simulink model "afe_dq_ttype"  (R2026b)
settings: Solver=ode23tb  StopTime=param.sim.simlength  FixedStep=param.sim.tc  MaxStep=param.glb_time.tc
values from neighbouring files (symbols this model uses):
  param = struct()    [init_model.m]
undefined symbols (not defined in the file or in its folder): magnitude
libraries: fl_lib x281, nesl_utility x136, igbt_simple_2th_lib x12, single_phase_transformer_lib x3, discrete_time_low_pass_filter x1, threephase_inductor_lib x1, dclink_for_three_levels x1, three_phase_three_level_ttype_inverter_ideal_switch_based_model x1, three_phase_three_levels_PWM_modulator x1, three_phase_bridge_three_level_ttype_igbt_simple_2th x1, three_phase_voltage_with_frt_emulator_mfcn x1
(part 2 of 8)

== system afe_dq_ttype/afe_dq_mod1/LCL_filter/threephase_vi_measures_stack1 ==
  Bus Creator : BusCreator  Inputs=6
  Current Sensor : fl_lib/Electrical/Electrical Sensors/Current Sensor
  Current Sensor1 : fl_lib/Electrical/Electrical Sensors/Current Sensor
  Current Sensor2 : fl_lib/Electrical/Electrical Sensors/Current Sensor
  Electrical Reference1 : fl_lib/Electrical/Electrical Elements/Electrical Reference
  Gain1 : Gain  Gain=1/param.afe.hw.ubez
  Gain2 : Gain  Gain=1/param.afe.hw.ubez
  Gain3 : Gain  Gain=1/param.afe.hw.ubez
  Gain4 : Gain  Gain=1/param.afe.hw.ibez
  Gain5 : Gain  Gain=1/param.afe.hw.ibez
  Gain6 : Gain  Gain=1/param.afe.hw.ibez
  Selector : Selector  InputPortWidth=6  IndexOptions=Index vector (dialog)  Indices=[1 2 3]  OutputSizes=1  RuntimeRangeChecks=off
  Selector1 : Selector  InputPortWidth=6  IndexOptions=Index vector (dialog)  Indices=[4 5 6]  OutputSizes=1  RuntimeRangeChecks=off
  Voltage Sensor : fl_lib/Electrical/Electrical Sensors/Voltage Sensor
  Voltage Sensor1 : fl_lib/Electrical/Electrical Sensors/Voltage Sensor
  Voltage Sensor2 : fl_lib/Electrical/Electrical Sensors/Voltage Sensor
  ia_grid : nesl_utility/PS-Simulink Converter  PhysicalDomain=network_engine_domain  SubClassName=ps_output  LeftPortType=input  RightPortType=output  PseudoPeriodic=off  Frequencies=[]  VectorFormat=1-D array  Unit=A  AffineConversion=off
  ib_grid : nesl_utility/PS-Simulink Converter  PhysicalDomain=network_engine_domain  SubClassName=ps_output  LeftPortType=input  RightPortType=output  PseudoPeriodic=off  Frequencies=[]  VectorFormat=1-D array  Unit=A  AffineConversion=off
  ic_grid : nesl_utility/PS-Simulink Converter  PhysicalDomain=network_engine_domain  SubClassName=ps_output  LeftPortType=input  RightPortType=output  PseudoPeriodic=off  Frequencies=[]  VectorFormat=1-D array  Unit=A  AffineConversion=off
  ua_grid : nesl_utility/PS-Simulink Converter  PhysicalDomain=network_engine_domain  SubClassName=ps_output  LeftPortType=input  RightPortType=output  PseudoPeriodic=off  Frequencies=[]  VectorFormat=1-D array  Unit=V  AffineConversion=off
  ub_grid : nesl_utility/PS-Simulink Converter  PhysicalDomain=network_engine_domain  SubClassName=ps_output  LeftPortType=input  RightPortType=output  PseudoPeriodic=off  Frequencies=[]  VectorFormat=1-D array  Unit=V  AffineConversion=off
  uc_grid : nesl_utility/PS-Simulink Converter  PhysicalDomain=network_engine_domain  SubClassName=ps_output  LeftPortType=input  RightPortType=output  PseudoPeriodic=off  Frequencies=[]  VectorFormat=1-D array  Unit=V  AffineConversion=off
  Ua : PMIOPort  Side=Left
  ua : PMIOPort  Port=2  Side=Right
  Ub : PMIOPort  Port=3  Side=Left
  ub : PMIOPort  Port=4  Side=Right
  Uc : PMIOPort  Port=5  Side=Left
  uc : PMIOPort  Port=6  Side=Right
  tag scope: ig_abc_pu_mod1=global, ug_abc_pu_mod1=global
  wires:
  Selector1/1 -> [ig_abc_pu_mod1]
  uc_grid/1 -> Gain3/1
  ub_grid/1 -> Gain2/1
  ua_grid/1 -> Gain1/1
  ic_grid/1 -> Gain5/1
  ia_grid/1 -> Gain6/1
  ib_grid/1 -> Gain4/1
  Selector/1 -> [ug_abc_pu_mod1]
  Bus Creator/1 -> Selector1/1, Selector/1  "vi_data"
  Gain1/1 -> Bus Creator/1  "ua_grid_pu"
  Gain2/1 -> Bus Creator/2  "ub_grid_pu"
  Gain3/1 -> Bus Creator/3  "uc_grid_pu"
  Gain6/1 -> Bus Creator/4  "ia_grid_pu"
  Gain4/1 -> Bus Creator/5  "ib_grid_pu"
  Gain5/1 -> Bus Creator/6  "ic_grid_pu"
  connections:
  Current Sensor2/RConn2 -- uc/RConn1
  ic_grid/LConn1 -- Current Sensor2/RConn1
  ia_grid/LConn1 -- Current Sensor/RConn1
  ib_grid/LConn1 -- Current Sensor1/RConn1
  Voltage Sensor2/RConn1 -- uc_grid/LConn1
  Current Sensor1/RConn2 -- ub/RConn1
  Voltage Sensor/LConn1 -- Current Sensor/LConn1 -- Ua/RConn1
  Current Sensor2/LConn1 -- Voltage Sensor2/LConn1 -- Uc/RConn1
  Voltage Sensor1/RConn1 -- ub_grid/LConn1
  Current Sensor/RConn2 -- ua/RConn1
  Voltage Sensor/RConn1 -- ua_grid/LConn1
  Voltage Sensor1/RConn2 -- Voltage Sensor2/RConn2 -- Voltage Sensor/RConn2 -- Electrical Reference1/LConn1
  Voltage Sensor1/LConn1 -- Current Sensor1/LConn1 -- Ub/RConn1

== system afe_dq_ttype/afe_dq_mod1/afe/deadtime_generator_for_ttype ==
  gate_cmds_in : Inport
  Bus Creator : BusCreator  Inputs=3
  dead_time_generator_cmos_simulink_phu : Subsystem  mask{ts=param.glb_time.tc, positive_voltage_rail=15, dead_time=param.glb_time.dead_time_AFE}
      mask prompts: ts "PT1 tau [s]"; positive_voltage_rail "Positive Voltage Rail [V]"; dead_time "DeadTime [s]"
  dead_time_generator_cmos_simulink_phv : Subsystem  mask{ts=param.glb_time.tc, positive_voltage_rail=15, dead_time=param.glb_time.dead_time_AFE}
      mask prompts: ts "PT1 tau [s]"; positive_voltage_rail "Positive Voltage Rail [V]"; dead_time "DeadTime [s]"
  dead_time_generator_cmos_simulink_phw : Subsystem  mask{ts=param.glb_time.tc, positive_voltage_rail=15, dead_time=param.glb_time.dead_time_AFE}
      mask prompts: ts "PT1 tau [s]"; positive_voltage_rail "Positive Voltage Rail [V]"; dead_time "DeadTime [s]"
  gate_cmds_out : Outport
  wires:
  Bus Creator/1 -> gate_cmds_out/1  "gate_cmds"
  dead_time_generator_cmos_simulink_phu/1(cmd_gates) -> Bus Creator/1  "gate_cmds_phu"
  gate_cmds_in/1 -> dead_time_generator_cmos_simulink_phu/1(gate_commands), dead_time_generator_cmos_simulink_phw/1(gate_commands), dead_time_generator_cmos_simulink_phv/1(gate_commands)
  dead_time_generator_cmos_simulink_phw/1(cmd_gates) -> Bus Creator/3  "gate_cmds_phw"
  dead_time_generator_cmos_simulink_phv/1(cmd_gates) -> Bus Creator/2  "gate_cmds_phv"

== system afe_dq_ttype/afe_dq_mod1/afe/ideal_switch_based_three_level_inverter_ttype ==
  gate_commands : Inport
  ideal_switch_based_three_level_inverter_ttype : three_phase_three_level_ttype_inverter_ideal_switch_based_model/ideal_switch_based_three_level_inverter_ttype  Vth=5.5  Ron=1.5e-3  Vdon_diode=2  Rdon_diode=0.15e-3  Csnubber=10e-9  Rsnubber=2200
  uu : PMIOPort  Side=Left
  uv : PMIOPort  Port=2  Side=Left
  udc(+) : PMIOPort  Port=3  Side=Right
  np : PMIOPort  Port=4  Side=Right
  udc(-) : PMIOPort  Port=5  Side=Right
  uw : PMIOPort  Port=6  Side=Left
  wires:
  gate_commands/1 -> ideal_switch_based_three_level_inverter_ttype/1
  connections:
  ideal_switch_based_three_level_inverter_ttype/RConn3 -- udc(-)/RConn1
  uv/RConn1 -- ideal_switch_based_three_level_inverter_ttype/LConn2
  ideal_switch_based_three_level_inverter_ttype/LConn1 -- uu/RConn1
  udc(+)/RConn1 -- ideal_switch_based_three_level_inverter_ttype/RConn1
  ideal_switch_based_three_level_inverter_ttype/LConn3 -- uw/RConn1
  ideal_switch_based_three_level_inverter_ttype/RConn2 -- np/RConn1

== system afe_dq_ttype/afe_dq_mod1/afe/igbt_based_three_level_three_phase_inverter_ttype ==
  gate_commands : Inport
  Bus Selector1 : BusSelector  OutputSignals=igbt_ploss_Q1,igbt_ploss_Q4,igbt_ploss_Q2,igbt_ploss_Q3  OutputAsBus=on
  Bus Selector2 : BusSelector  OutputSignals=diode_ploss_Q4,diode_ploss_Q3,diode_ploss_Q2,diode_ploss_Q1  OutputAsBus=on
  diode_plosses : Scope
      settings: ActiveDisplayYMinimum=-84.335211962463276  ActiveDisplayYMaximum=759.01696526250635  DataLoggingVariableName=ScopeData3
  igbt_plosses : Scope
      settings: ActiveDisplayYMinimum=-229.25636650117849  ActiveDisplayYMaximum=1454.3450749918761
  three_phase_inverter_igbt_2th_based_ttype : Subsystem  mask{Vth_inv_t_m=param.afe.igbt.Vth, Vce_sat_inv_t_m=param.afe.igbt.Vce_sat, Rce_on_inv_t_m=param.afe.igbt.Rce_on, Eon_inv_t_m=param.afe.igbt.Eon, Eoff_inv_t_m=param.afe.igbt.Eoff, Erec_inv_t_m=param.afe.igbt.Erec, Ion_sw_loss_inv_t_m=param.afe.igbt.Ion_sw_losses, Voff_sw_loss_inv_t_m=param.afe.igbt.Voff_sw_losses, Vdon_diode_inv_t_m=param.afe.igbt.Vdon_diode, Rdon_diode_inv_t_m=param.afe.igbt.Rdon_diode, rth_switch_JH_inv_t_m=param.afe.igbt.Rth_switch_JH, rth_switch_HA_inv_t_m=param.thermal.heatsink.Rth_switch_HA, rth_diode_JH_inv_t_m=param.afe.igbt.Rth_diode_JH, rth_diode_HA_inv_t_m=param.thermal.heatsink.Rth_diode_HA, Csnubber_inv_t_m=param.afe.igbt.Csnubber, Rsnubber_inv_t_m=param.afe.igbt.Rsnubber, Vth_m=param.afe.igbt.Vth, Vce_sat_m=param.afe.igbt.Vce_sat, Rce_on_m=param.afe.igbt.Rce_on, Eon_m=param.afe.igbt.Eon, Eoff_m=param.afe.igbt.Eoff, Erec_m=param.afe.igbt.Erec, Ion_sw_loss_m=param.afe.igbt.Ion_sw_losses, Voff_sw_loss_m=param.afe.igbt.Voff_sw_losses, Vdon_diode_m=param.afe.igbt.Vdon_diode, Rdon_diode_m=param.afe.igbt.Rdon_diode, rth_switch_JH_m=param.afe.igbt.Rth_switch_JH, rth_switch_HA_m=param.thermal.heatsink.Rth_switch_HA, rth_diode_JH_m=param.afe.igbt.Rth_diode_JH, rth_diode_HA_m=param.thermal.heatsink.Rth_diode_HA, Csnubber_m=param.afe.igbt.Csnubber, Rsnubber_m=param.afe.igbt.Rsnubber, JunctionTermalMass_m=param.afe.igbt.JunctionTermalMass, mass_heatsink_m=param.thermal.heatsink.no_weight, specific_heat_m=param.thermal.heatsink.cp, Tambient_m=param.thermal.heatsink.Tambient, DThs_init_m=param.thermal.heatsink.DThs_init, tc_m=param.glb_time.tc}
      mask prompts: Vth_inv_t_m "Vth (V)"; Vce_sat_inv_t_m "Vce_sat (V)"; Rce_on_inv_t_m "Rce_on (Ohm)"; Eon_inv_t_m "Eon (J)"; Eoff_inv_t_m "Eoff (J)"; Erec_inv_t_m "Erec (J)"; Ion_sw_loss_inv_t_m "Ion_sw_loss (A)"; Voff_sw_loss_inv_t_m "Voff_sw_loss (V)"; Vdon_diode_inv_t_m "Vdon_diode (V)"; Rdon_diode_inv_t_m "Rdon_diode (Ohm)"; rth_switch_JH_inv_t_m "rth_switch_JH (K/W)"; rth_switch_HA_inv_t_m "rth_switch_HA  (K/W)"; rth_diode_JH_inv_t_m "rth_diode_JH (K/W)"; rth_diode_HA_inv_t_m "rth_diode_HA  (K/W)"; Csnubber_inv_t_m "Csnubber (F)"; Rsnubber_inv_t_m "Rsnubber (Ohm)"; Vth_m "Vth (V)"; Vce_sat_m "Vce_sat (V)"; Rce_on_m "Rce_on (Ohm)"; Eon_m "Eon (J)"; Eoff_m "Eoff (J)"; Erec_m "Erec (J)"; Ion_sw_loss_m "Ion_sw_loss (A)"; Voff_sw_loss_m "Voff_sw_loss (V)"; Vdon_diode_m "Vdon_diode (V)"; Rdon_diode_m "Rdon_diode (Ohm)"; rth_switch_JH_m "rth_switch_JH (K/W)"; rth_switch_HA_m "rth_switch_HA  (K/W)"; rth_diode_JH_m "rth_diode_JH (K/W)"; rth_diode_HA_m "rth_diode_HA  (K/W)"; Csnubber_m "Csnubber (F)"; Rsnubber_m "Rsnubber (Ohm)"; JunctionTermalMass_m "JunctionTermalMass (J/K)"; mass_heatsink_m "mass_heatsink (Kg)"; specific_heat_m "specific_heat (J/(K*Kg))"; Tambient_m "Tambient (Celsius)"; DThs_init_m "DThs_init (Celsius)"; tc_m "tc"
      mask DialogControl inv_t Prompt: T-IGBT
      mask DialogControl inv Prompt: IGBT
      mask DialogControl thermal Prompt: Thermal
      mask DialogControl solver Prompt: Solver
  udc(+) : PMIOPort  Side=Right
  uu : PMIOPort  Port=2  Side=Left
  np : PMIOPort  Port=3  Side=Right
  uv : PMIOPort  Port=4  Side=Left
  udc(-) : PMIOPort  Port=5  Side=Right
  uw : PMIOPort  Port=6  Side=Left
  wires:
  Bus Selector2/1 -> diode_plosses/1
  Bus Selector1/1 -> igbt_plosses/1
  three_phase_inverter_igbt_2th_based_ttype/1(m) -> Bus Selector1/1, Bus Selector2/1
  gate_commands/1 -> three_phase_inverter_igbt_2th_based_ttype/1(gate_commands)
  connections:
  three_phase_inverter_igbt_2th_based_ttype/RConn1 -- udc(+)/RConn1
  three_phase_inverter_igbt_2th_based_ttype/LConn1 -- uu/RConn1
  three_phase_inverter_igbt_2th_based_ttype/LConn3 -- uw/RConn1
  three_phase_inverter_igbt_2th_based_ttype/LConn2 -- uv/RConn1
  three_phase_inverter_igbt_2th_based_ttype/RConn3 -- udc(-)/RConn1
  three_phase_inverter_igbt_2th_based_ttype/RConn2 -- np/RConn1

== system afe_dq_ttype/afe_dq_mod1/afe/sv_pwm ==
  duties_uvw : Inport
  Bus Selector2 : BusSelector  OutputSignals=du(k),dv(k),dw(k)
  Constant1 : Constant  Value=param.afe.behav.pwm_phase_shift_mod1
  modulator1 : Subsystem
  td2tc_1 : TransferFcn  Denominator=[param.glb_time.tc 1]
  td2tc_2 : TransferFcn  Denominator=[param.glb_time.tc 1]
  td2tc_3 : TransferFcn  Denominator=[param.glb_time.tc 1]
  gate_cmds : Outport
  wires:
  modulator1/1(gate_cmds) -> gate_cmds/1
  Constant1/1 -> modulator1/4(phase)
  Bus Selector2/1 -> td2tc_1/1  "<du(k)>"
  Bus Selector2/2 -> td2tc_2/1  "<dv(k)>"
  Bus Selector2/3 -> td2tc_3/1  "<dw(k)>"
  duties_uvw/1 -> Bus Selector2/1
  td2tc_1/1 -> modulator1/1(u)  "du(t)"
  td2tc_3/1 -> modulator1/3(w)  "dw(t)"
  td2tc_2/1 -> modulator1/2(v)  "dv(t)"

== system afe_dq_ttype/afe_dq_mod1/afe/three_phase_bridge_three_level_ttype_igbt_simple_2th ==
  gate_cmds : Inport
  Bus Selector1 : BusSelector  OutputSignals=igbt_ploss_Q1,igbt_ploss_Q4,igbt_ploss_Q2,igbt_ploss_Q3  OutputAsBus=on
  Bus Selector2 : BusSelector  OutputSignals=diode_ploss_Q4,diode_ploss_Q3,diode_ploss_Q2,diode_ploss_Q1  OutputAsBus=on
  diode_plosses : Scope
      settings: ActiveDisplayYMinimum=-101.38535998641856  ActiveDisplayYMaximum=912.4682991261559  DataLoggingVariableName=ScopeData5
  igbt_plosses : Scope
      settings: ActiveDisplayYMinimum=-571.07488373842511  ActiveDisplayYMaximum=5139.6739536458181  DataLoggingVariableName=ScopeData6
  three_phase_bridge_three_level_ttype_igbt_simple_2th : three_phase_bridge_three_level_ttype_igbt_simple_2th/three_phase_bridge_three_level_ttype_igbt_simple_2th  vce_sat_m=param.afe.igbt.Vce_sat  rce_on_m=param.afe.igbt.Rce_on  v_gamma_m=param.afe.igbt.Vdon_diode  rd_on_m=param.afe.igbt.Rdon_diode  Gce_off_m=1e-6  Vth_gate_m=param.afe.igbt.Vth  Vth_gate_hyst_m=0.85  Eon_m=param.afe.igbt.Eon*1000  Eoff_m=param.afe.igbt.Eoff*1000  Err_m=param.afe.igbt.Erec*1000  Ic_ref_m=param.afe.igbt.Ion_sw_losses  Vdc_ref_m=param.afe.igbt.Voff_sw_losses  Vblock_Errf_m=50  time_constant_edge_m=param.glb_time.tc*1e6  time_constant_ploss_m=param.glb_time.tPWM_AFE*5*1e6  Csnubber_m=12e-12  Rsnubber_m=2200  rth_switch_JH_m=param.afe.igbt.Rth_switch_JH  rth_switch_HA_m=param.thermal.Rth_switch_HA  rth_diode_JH_m=param.afe.igbt.Rth_diode_JH  rth_diode_HA_m=param.thermal.Rth_diode_HA  JunctionTermalMass_m=param.afe.igbt.JunctionTermalMass  Tambient_m=param.thermal.Tambient  mass_heatsink_m=param.thermal.weight  specific_heat_m=param.thermal.cp_al
  udc(+) : PMIOPort  Side=Left
  np : PMIOPort  Port=2  Side=Left
  udc(-) : PMIOPort  Port=3  Side=Left
  u : PMIOPort  Port=4  Side=Right
  v : PMIOPort  Port=5  Side=Right
  w : PMIOPort  Port=6  Side=Right
  wires:
  gate_cmds/1 -> three_phase_bridge_three_level_ttype_igbt_simple_2th/1
  three_phase_bridge_three_level_ttype_igbt_simple_2th/1 -> Bus Selector1/1, Bus Selector2/1
  Bus Selector1/1 -> igbt_plosses/1
  Bus Selector2/1 -> diode_plosses/1
  connections:
  np/RConn1 -- three_phase_bridge_three_level_ttype_igbt_simple_2th/LConn2
  three_phase_bridge_three_level_ttype_igbt_simple_2th/RConn1 -- u/RConn1
  udc(+)/RConn1 -- three_phase_bridge_three_level_ttype_igbt_simple_2th/LConn1
  udc(-)/RConn1 -- three_phase_bridge_three_level_ttype_igbt_simple_2th/LConn3
  three_phase_bridge_three_level_ttype_igbt_simple_2th/RConn2 -- v/RConn1
  three_phase_bridge_three_level_ttype_igbt_simple_2th/RConn3 -- w/RConn1

== system afe_dq_ttype/grid/grid_emulator/3ph_Dyg ==
  Electrical Reference1 : fl_lib/Electrical/Electrical Elements/Electrical Reference
  ph1 : single_phase_transformer_lib/single phase transformer  Lm=param.grid.emu.trafo.Lm1 H  n1=param.grid.emu.trafo.n1  n2=param.grid.emu.trafo.n2  Rd1=param.grid.emu.trafo.Rd1 Ohm  Rd2=param.grid.emu.trafo.Rd2 Ohm  Ld1=param.grid.emu.trafo.Ld1 H  Ld2=param.grid.emu.trafo.Ld2 H  Rfe=param.grid.emu.trafo.Rfe1 Ohm  phi_specify=off  phi_priority=None  phi=0 V*s  phi_nominal_specify=off  phi_nominal_value=1  phi_nominal_unit=V*s  i1_specify=off  i1_priority=None  i1=0 A  i1_nominal_specify=off  i1_nominal_value=1  i1_nominal_unit=A  i2_specify=off  i2_priority=None  i2=0 A  i2_nominal_specify=off  i2_nominal_value=1  i2_nominal_unit=A  ife_specify=off  ife_priority=None  ife=0 A  ife_nominal_specify=off  ife_nominal_value=1  ife_nominal_unit=A  u1_specify=off  u1_priority=None  u1=0 V  u1_nominal_specify=off  u1_nominal_value=1  u1_nominal_unit=V  u2_specify=off  u2_priority=None  u2=0 V  u2_nominal_specify=off  u2_nominal_value=1  u2_nominal_unit=V
  ph2 : single_phase_transformer_lib/single phase transformer  Lm=param.grid.emu.trafo.Lm1 H  n1=param.grid.emu.trafo.n1  n2=param.grid.emu.trafo.n2  Rd1=param.grid.emu.trafo.Rd1 Ohm  Rd2=param.grid.emu.trafo.Rd2 Ohm  Ld1=param.grid.emu.trafo.Ld1 H  Ld2=param.grid.emu.trafo.Ld2 H  Rfe=param.grid.emu.trafo.Rfe1 Ohm  phi_specify=off  phi_priority=None  phi=0 V*s  phi_nominal_specify=off  phi_nominal_value=1  phi_nominal_unit=V*s  i1_specify=off  i1_priority=None  i1=0 A  i1_nominal_specify=off  i1_nominal_value=1  i1_nominal_unit=A  i2_specify=off  i2_priority=None  i2=0 A  i2_nominal_specify=off  i2_nominal_value=1  i2_nominal_unit=A  ife_specify=off  ife_priority=None  ife=0 A  ife_nominal_specify=off  ife_nominal_value=1  ife_nominal_unit=A  u1_specify=off  u1_priority=None  u1=0 V  u1_nominal_specify=off  u1_nominal_value=1  u1_nominal_unit=V  u2_specify=off  u2_priority=None  u2=0 V  u2_nominal_specify=off  u2_nominal_value=1  u2_nominal_unit=V
  ph3 : single_phase_transformer_lib/single phase transformer  Lm=param.grid.emu.trafo.Lm1 H  n1=param.grid.emu.trafo.n1  n2=param.grid.emu.trafo.n2  Rd1=param.grid.emu.trafo.Rd1 Ohm  Rd2=param.grid.emu.trafo.Rd2 Ohm  Ld1=param.grid.emu.trafo.Ld1 H  Ld2=param.grid.emu.trafo.Ld2 H  Rfe=param.grid.emu.trafo.Rfe1 Ohm  phi_specify=off  phi_priority=None  phi=0 V*s  phi_nominal_specify=off  phi_nominal_value=1  phi_nominal_unit=V*s  i1_specify=off  i1_priority=None  i1=0 A  i1_nominal_specify=off  i1_nominal_value=1  i1_nominal_unit=A  i2_specify=off  i2_priority=None  i2=0 A  i2_nominal_specify=off  i2_nominal_value=1  i2_nominal_unit=A  ife_specify=off  ife_priority=None  ife=0 A  ife_nominal_specify=off  ife_nominal_value=1  ife_nominal_unit=A  u1_specify=off  u1_priority=None  u1=0 V  u1_nominal_specify=off  u1_nominal_value=1  u1_nominal_unit=V  u2_specify=off  u2_priority=None  u2=0 V  u2_nominal_specify=off  u2_nominal_value=1  u2_nominal_unit=V
  ua : PMIOPort  Side=Right
  ub : PMIOPort  Port=2  Side=Right
  uc : PMIOPort  Port=3  Side=Right
  Ua : PMIOPort  Port=4  Side=Left
  Ub : PMIOPort  Port=5  Side=Left
  Uc : PMIOPort  Port=6  Side=Left
  connections:
  Electrical Reference1/LConn1 -- ph3/RConn2 -- ph2/RConn2 -- ph1/RConn2
  ph3/RConn1 -- uc/RConn1
  ph1/LConn1 -- ph3/LConn2 -- Ua/RConn1
  ph1/RConn1 -- ua/RConn1
  ph2/RConn1 -- ub/RConn1
  ph1/LConn2 -- ph2/LConn1 -- Ub/RConn1
  Uc/RConn1 -- ph3/LConn1 -- ph2/LConn2

== system afe_dq_ttype/grid/grid_emulator/threephase_vi_measures ==
  Bus Creator : BusCreator  Inputs=6
  Current Sensor : fl_lib/Electrical/Electrical Sensors/Current Sensor
  Current Sensor1 : fl_lib/Electrical/Electrical Sensors/Current Sensor
  Current Sensor2 : fl_lib/Electrical/Electrical Sensors/Current Sensor
  Electrical Reference1 : fl_lib/Electrical/Electrical Elements/Electrical Reference
  Voltage Sensor : fl_lib/Electrical/Electrical Sensors/Voltage Sensor
  Voltage Sensor1 : fl_lib/Electrical/Electrical Sensors/Voltage Sensor
  Voltage Sensor2 : fl_lib/Electrical/Electrical Sensors/Voltage Sensor
  i : Selector  InputPortWidth=6  IndexOptions=Index vector (dialog)  Indices=[4 5 6]  OutputSizes=1  RuntimeRangeChecks=off
  ia_grid : nesl_utility/PS-Simulink Converter  PhysicalDomain=network_engine_domain  SubClassName=ps_output  LeftPortType=input  RightPortType=output  PseudoPeriodic=off  Frequencies=[]  VectorFormat=1-D array  Unit=A  AffineConversion=off
  ib_grid : nesl_utility/PS-Simulink Converter  PhysicalDomain=network_engine_domain  SubClassName=ps_output  LeftPortType=input  RightPortType=output  PseudoPeriodic=off  Frequencies=[]  VectorFormat=1-D array  Unit=A  AffineConversion=off
  ic_grid : nesl_utility/PS-Simulink Converter  PhysicalDomain=network_engine_domain  SubClassName=ps_output  LeftPortType=input  RightPortType=output  PseudoPeriodic=off  Frequencies=[]  VectorFormat=1-D array  Unit=A  AffineConversion=off
  u : Selector  InputPortWidth=6  IndexOptions=Index vector (dialog)  Indices=[1 2 3]  OutputSizes=1  RuntimeRangeChecks=off
  ua_grid : nesl_utility/PS-Simulink Converter  PhysicalDomain=network_engine_domain  SubClassName=ps_output  LeftPortType=input  RightPortType=output  PseudoPeriodic=off  Frequencies=[]  VectorFormat=1-D array  Unit=V  AffineConversion=off
  ub_grid : nesl_utility/PS-Simulink Converter  PhysicalDomain=network_engine_domain  SubClassName=ps_output  LeftPortType=input  RightPortType=output  PseudoPeriodic=off  Frequencies=[]  VectorFormat=1-D array  Unit=V  AffineConversion=off
  uc_grid : nesl_utility/PS-Simulink Converter  PhysicalDomain=network_engine_domain  SubClassName=ps_output  LeftPortType=input  RightPortType=output  PseudoPeriodic=off  Frequencies=[]  VectorFormat=1-D array  Unit=V  AffineConversion=off
  Ua : PMIOPort  Side=Left
  ua : PMIOPort  Port=2  Side=Right
  Ub : PMIOPort  Port=3  Side=Left
  ub : PMIOPort  Port=4  Side=Right
  Uc : PMIOPort  Port=5  Side=Left
  uc : PMIOPort  Port=6  Side=Right
  tag scope: i_abc_line=global, u_abc_line=global
  wires:
  Bus Creator/1 -> i/1, u/1  "vi_data"
  ib_grid/1 -> Bus Creator/5  "ib"
  ia_grid/1 -> Bus Creator/4  "ia"
  ic_grid/1 -> Bus Creator/6  "ic"
  ua_grid/1 -> Bus Creator/1  "ua"
  ub_grid/1 -> Bus Creator/2  "ub"
  uc_grid/1 -> Bus Creator/3  "uc"
  i/1 -> [i_abc_line]
  u/1 -> [u_abc_line]
  connections:
  Current Sensor1/LConn1 -- Ub/RConn1 -- Voltage Sensor1/LConn1
  Electrical Reference1/LConn1 -- Voltage Sensor/RConn2 -- Voltage Sensor2/RConn2 -- Voltage Sensor1/RConn2
  Voltage Sensor/RConn1 -- ua_grid/LConn1
  Current Sensor/RConn2 -- ua/RConn1
  Voltage Sensor1/RConn1 -- ub_grid/LConn1
  Voltage Sensor2/LConn1 -- Current Sensor2/LConn1 -- Uc/RConn1
  Current Sensor/LConn1 -- Ua/RConn1 -- Voltage Sensor/LConn1
  Current Sensor1/RConn2 -- ub/RConn1
  Voltage Sensor2/RConn1 -- uc_grid/LConn1
  ib_grid/LConn1 -- Current Sensor1/RConn1
  ia_grid/LConn1 -- Current Sensor/RConn1
  ic_grid/LConn1 -- Current Sensor2/RConn1
  Current Sensor2/RConn2 -- uc/RConn1

== system afe_dq_ttype/afe_dq_mod1/AFE_control/afe_control/acquisitions ==
  ug_abc_pu : Inport
  udc_pu : Inport  Port=2
  ig_abc_pu : Inport  Port=3
  is_abc_pu : Inport  Port=4
  master_time : Inport  Port=5
  grid_phase : Inport  Port=6
  Terminator : Terminator
  grid_phase_acquisition : Subsystem
  ig afe quantizzation and one step delay : Subsystem
  is afe quantizzation and one step delay : Subsystem
  phase_compensation_1 : Subsystem
  udc_acquisition : Subsystem
  ug afe quantizzation and one step delay : Subsystem
  AFE1_local_time_corr : Outport
  tag scope: grid_emulator_phase=scoped, igd_abc_pu=scoped, isd_abc_pu=scoped, udcd_pu_afe=scoped, ugd_abc_pu=scoped
  wires:
  grid_phase/1 -> grid_phase_acquisition/1(grid_phase)
  grid_phase_acquisition/1(grid_phased) -> [grid_emulator_phase]
  udc_acquisition/1(udcd_pu) -> [udcd_pu_afe]
  ig_abc_pu/1 -> ig afe quantizzation and one step delay/1(ig_abc_pu)
  ug_abc_pu/1 -> ug afe quantizzation and one step delay/1(ug_abc_pu)
  [udcd_pu_afe] -> Terminator/1
  phase_compensation_1/1(y) -> AFE1_local_time_corr/1
  is_abc_pu/1 -> is afe quantizzation and one step delay/1(is_abc_pu)
  master_time/1 -> phase_compensation_1/2(master_time)
  udc_pu/1 -> udc_acquisition/1(udc_pu)
  ig afe quantizzation and one step delay/1(igd_abc_pu) -> [igd_abc_pu]
  [local_time] -> phase_compensation_1/1(local_time)
  is afe quantizzation and one step delay/1(isd_abc_pu) -> [isd_abc_pu]
  ug afe quantizzation and one step delay/1(ugd_abc_pu) -> [ugd_abc_pu]

== system afe_dq_ttype/afe_dq_mod1/AFE_control/afe_control/current_ctrl ==
  i_xi_ref : Inport
  Constant : Constant  Value=0
  Demux : Demux  Outputs=3
  current_transformation : Subsystem
  dq_vector_pi : Subsystem
  xi_eta_to_alpha_beta : MATLAB Function  TreatAsAtomicUnit=on
  zero_current_ctrl : Subsystem
  uabg : Outport  VectorParamsAs1DForOutWhenUnconnected=off
  wires:
  Demux/1 -> current_transformation/1(is_a_pu)  "is_a"
  Demux/2 -> current_transformation/2(is_b_pu)  "is_b"
  Demux/3 -> current_transformation/3(is_c_pu)  "is_c"
  [isd_abc_pu] -> Demux/1
  [phase_grid_pll] -> xi_eta_to_alpha_beta/3(phase)
  [id_xi_pu] -> dq_vector_pi/1(id)
  [id_eta_pu] -> dq_vector_pi/3(iq)
  i_xi_ref/1 -> dq_vector_pi/2(id_ref)
  Constant/1 -> dq_vector_pi/4(iq_ref)
  zero_current_ctrl/1(uabg_ctrl_out) -> uabg/1
  dq_vector_pi/1(md_sat) -> xi_eta_to_alpha_beta/1(xi)
  dq_vector_pi/2(mq_sat) -> xi_eta_to_alpha_beta/2(eta)
  xi_eta_to_alpha_beta/1(alpha) -> zero_current_ctrl/1(ualpha_ctrl_afe)
  xi_eta_to_alpha_beta/2(beta) -> zero_current_ctrl/2(ubeta_ctrl_afe)

== system afe_dq_ttype/afe_dq_mod1/AFE_control/afe_control/data_to_worspace_module_1 ==
  Bus Creator : BusCreator  Inputs=3
  dq_pll : Subsystem
  pwr_meter : Subsystem
  m : Outport
  wires:
  Bus Creator/1 -> m/1
  pwr_meter/1(m_pwr_meter) -> Bus Creator/1  "pwr_meter"
  dq_pll/1(dqPLLs) -> Bus Creator/2  "dq_pll"
  [local_time] -> Bus Creator/3  "local_time"

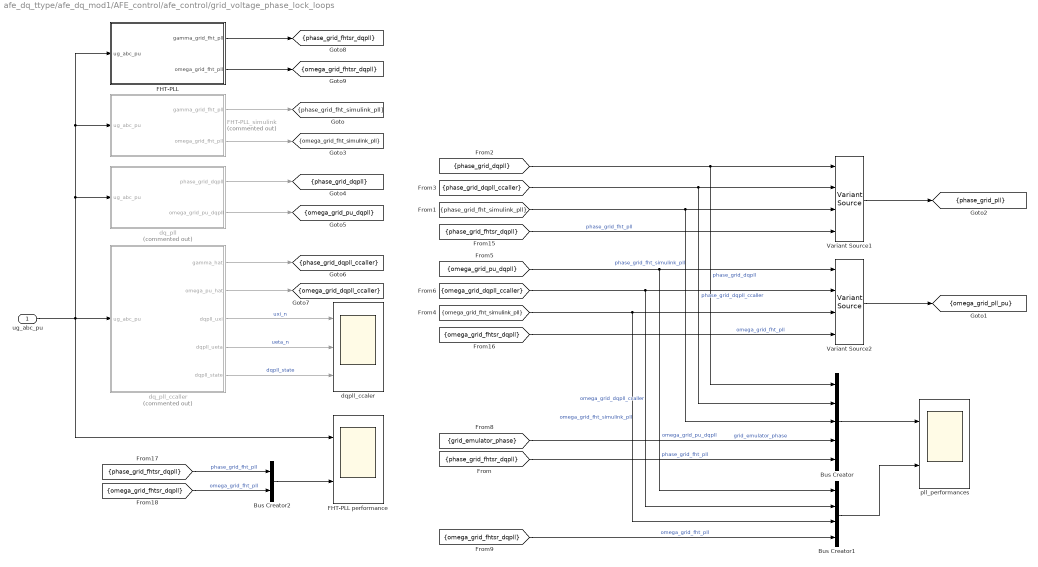
== system afe_dq_ttype/afe_dq_mod1/AFE_control/afe_control/grid_voltage_phase_lock_loops ==
  ug_abc_pu : Inport
  Bus Creator : BusCreator  Inputs=5
  Bus Creator1 : BusCreator  Inputs=4
  Bus Creator2 : BusCreator  Inputs=2
  FHT-PLL : Subsystem
  FHT-PLL performance : Scope  NumInputPorts=2
      settings: ActiveDisplayYMinimum=-1.251220703125  ActiveDisplayYMaximum=1.251220703125  DataLoggingVariableName=ScopeData8
  FHT-PLL_simulink : Subsystem  Commented=on
  Variant Source1 : VariantSource  VariantControls={param.afe.variant.dq_pll_mode1 == 1, param.afe.variant.dq_pll_mode2 == 1, param.afe.variant.dq_pll_mode3 == 1, param.afe.variant.dq_pll_mode4 == 1}
  Variant Source2 : VariantSource  VariantControls={param.afe.variant.dq_pll_mode1 == 1, param.afe.variant.dq_pll_mode2 == 1, param.afe.variant.dq_pll_mode3 == 1, param.afe.variant.dq_pll_mode4 == 1}
  dq_pll : Subsystem  Commented=on
  dq_pll_ccaller : Subsystem  Commented=on
  dqpll_ccaler : Scope  NumInputPorts=3
      settings: ActiveDisplayYMinimum=-0.88802937790751446  ActiveDisplayYMaximum=4.5431143753230572  DataLoggingVariableName=ScopeData4
  pll_performances : Scope  NumInputPorts=2
      settings: ActiveDisplayYMinimum=-3.9264641704366507  ActiveDisplayYMaximum=3.9264746341683896  DataLoggingVariableName=ScopeData34
  tag scope: omega_grid_dqpll_ccaller=scoped, omega_grid_fht_simulink_pll=scoped, omega_grid_fhtsr_dqpll=scoped, omega_grid_pll_pu=scoped, omega_grid_pu_dqpll=scoped, phase_grid_dqpll=scoped, phase_grid_dqpll_ccaller=scoped, phase_grid_fht_simulink_pll=scoped, phase_grid_fhtsr_dqpll=scoped, phase_grid_pll=scoped
  wires:
  Variant Source1/1 -> [phase_grid_pll]
  FHT-PLL_simulink/1(gamma_grid_fht_pll) -> [phase_grid_fht_simulink_pll]
  FHT-PLL_simulink/2(omega_grid_fht_pll) -> [omega_grid_fht_simulink_pll]
  dq_pll/2(omega_grid_pu_dqpll) -> [omega_grid_pu_dqpll]
  dq_pll/1(phase_grid_dqpll) -> [phase_grid_dqpll]
  dq_pll_ccaller/1(gamma_hat) -> [phase_grid_dqpll_ccaller]
  dq_pll_ccaller/2(omega_pu_hat) -> [omega_grid_dqpll_ccaller]
  [phase_grid_dqpll] -> Variant Source1/1, Bus Creator/1  "phase_grid_dqpll"
  [phase_grid_dqpll_ccaller] -> Bus Creator/2, Variant Source1/2  "phase_grid_dqpll_ccaller"
  [phase_grid_fht_simulink_pll] -> Bus Creator/3, Variant Source1/3  "phase_grid_fht_simulink_pll"
  [omega_grid_pu_dqpll] -> Variant Source2/1, Bus Creator1/1  "omega_grid_pu_dqpll"
  [omega_grid_dqpll_ccaller] -> Variant Source2/2, Bus Creator1/2  "omega_grid_dqpll_ccaller"
  [omega_grid_fht_simulink_pll] -> Variant Source2/3, Bus Creator1/3  "omega_grid_fht_simulink_pll"
  Variant Source2/1 -> [omega_grid_pll_pu]
  dq_pll_ccaller/3(dqpll_uxi) -> dqpll_ccaler/1  "uxi_n"
  dq_pll_ccaller/4(dqpll_ueta) -> dqpll_ccaler/2  "ueta_n"
  dq_pll_ccaller/5(dqpll_state) -> dqpll_ccaler/3  "dqpll_state"
  ug_abc_pu/1 -> FHT-PLL performance/1, dq_pll/1(ug_abc_pu), FHT-PLL_simulink/1(ug_abc_pu), FHT-PLL/1(ug_abc_pu), dq_pll_ccaller/1(ug_abc_pu)
  Bus Creator/1 -> pll_performances/1
  Bus Creator1/1 -> pll_performances/2
  [grid_emulator_phase] -> Bus Creator/4  "grid_emulator_phase"
  FHT-PLL/2(omega_grid_fht_pll) -> [omega_grid_fhtsr_dqpll]
  FHT-PLL/1(gamma_grid_fht_pll) -> [phase_grid_fhtsr_dqpll]
  [phase_grid_fhtsr_dqpll] -> Bus Creator/5  "phase_grid_fht_pll"
  [omega_grid_fhtsr_dqpll] -> Bus Creator1/4  "omega_grid_fht_pll"
  [phase_grid_fhtsr_dqpll] -> Variant Source1/4  "phase_grid_fht_pll"
  [omega_grid_fhtsr_dqpll] -> Variant Source2/4  "omega_grid_fht_pll"
  Bus Creator2/1 -> FHT-PLL performance/2
  [omega_grid_fhtsr_dqpll] -> Bus Creator2/2  "omega_grid_fht_pll"
  [phase_grid_fhtsr_dqpll] -> Bus Creator2/1  "phase_grid_fht_pll"

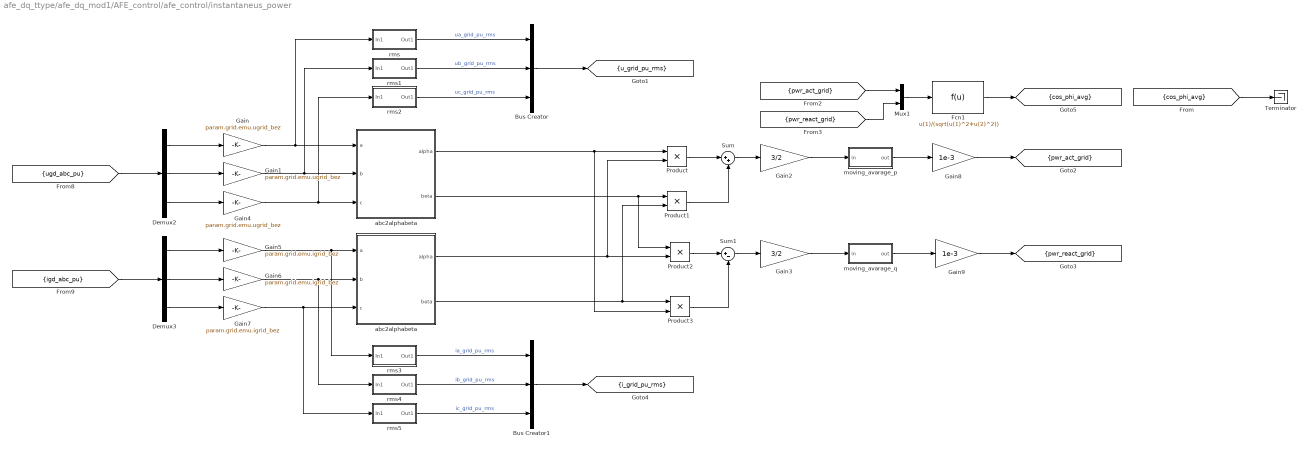
== system afe_dq_ttype/afe_dq_mod1/AFE_control/afe_control/instantaneus_power ==
  Bus Creator : BusCreator  Inputs=3
  Bus Creator1 : BusCreator  Inputs=3
  Demux2 : Demux  Outputs=3
  Demux3 : Demux  Outputs=3
  Fcn1 : Fcn  Expr=u(1)/(sqrt(u(1)^2+u(2)^2))
  Gain : Gain  Gain=param.grid.emu.ugrid_bez
  Gain1 : Gain  Gain=param.grid.emu.ugrid_bez
  Gain2 : Gain  Gain=3/2
  Gain3 : Gain  Gain=3/2
  Gain4 : Gain  Gain=param.grid.emu.ugrid_bez
  Gain5 : Gain  Gain=param.grid.emu.igrid_bez
  Gain6 : Gain  Gain=param.grid.emu.igrid_bez
  Gain7 : Gain  Gain=param.grid.emu.igrid_bez
  Gain8 : Gain  Gain=1e-3
  Gain9 : Gain  Gain=1e-3
  Mux1 : Mux  Inputs=2
  Product{,1..3} (4 alike) : Product  RndMeth=Zero
  Sum : Sum  Inputs=|++
  Sum1 : Sum  Inputs=|+-
  Terminator : Terminator
  abc2alphabeta : Subsystem
  "abc2alphabeta " : Subsystem
  moving_avarage_p : Subsystem
  moving_avarage_q : Subsystem
  rms : Subsystem
  rms1 : Subsystem
  rms2 : Subsystem
  rms3 : Subsystem
  rms4 : Subsystem
  rms5 : Subsystem
  tag scope: cos_phi_avg=scoped, i_grid_pu_rms=scoped, pwr_act_grid=scoped, pwr_react_grid=scoped, u_grid_pu_rms=scoped
  wires:
  abc2alphabeta/2("beta ") -> Product1/1, Product2/1
  "abc2alphabeta "/2("beta ") -> Product1/2, Product3/1
  abc2alphabeta/1("alpha ") -> Product3/2, Product/1
  "abc2alphabeta "/1("alpha ") -> Product2/2, Product/2
  Product/1 -> Sum/1
  Product1/1 -> Sum/2
  Product2/1 -> Sum1/1
  Product3/1 -> Sum1/2
  Sum1/1 -> Gain3/1
  Sum/1 -> Gain2/1
  Gain2/1 -> moving_avarage_p/1(in)
  Gain3/1 -> moving_avarage_q/1(in)
  [pwr_react_grid] -> Mux1/2
  Mux1/1 -> Fcn1/1
  Fcn1/1 -> [cos_phi_avg]
  [pwr_act_grid] -> Mux1/1
  rms/1(Out1) -> Bus Creator/1  "ua_grid_pu_rms"
  rms2/1(Out1) -> Bus Creator/3  "uc_grid_pu_rms"
  rms1/1(Out1) -> Bus Creator/2  "ub_grid_pu_rms"
  moving_avarage_p/1(out) -> Gain8/1
  moving_avarage_q/1(out) -> Gain9/1
  Demux2/1 -> Gain/1
  Demux2/2 -> Gain1/1
  Demux2/3 -> Gain4/1
  Demux3/1 -> Gain5/1
  Demux3/2 -> Gain6/1
  Demux3/3 -> Gain7/1
  Gain/1 -> rms/1(In1), abc2alphabeta/1(a)
  Gain1/1 -> rms1/1(In1), abc2alphabeta/2(b)
  Gain4/1 -> rms2/1(In1), abc2alphabeta/3(c)
  Gain5/1 -> rms3/1(In1), "abc2alphabeta "/1(a)
  Gain6/1 -> rms4/1(In1), "abc2alphabeta "/2(b)
  Gain7/1 -> rms5/1(In1), "abc2alphabeta "/3(c)
  Gain8/1 -> [pwr_act_grid]
  Gain9/1 -> [pwr_react_grid]
  [ugd_abc_pu] -> Demux2/1
  [igd_abc_pu] -> Demux3/1
  Bus Creator/1 -> [u_grid_pu_rms]
  rms4/1(Out1) -> Bus Creator1/2  "ib_grid_pu_rms"
  rms3/1(Out1) -> Bus Creator1/1  "ia_grid_pu_rms"
  rms5/1(Out1) -> Bus Creator1/3  "ic_grid_pu_rms"
  Bus Creator1/1 -> [i_grid_pu_rms]
  [cos_phi_avg] -> Terminator/1

== system afe_dq_ttype/afe_dq_mod1/AFE_control/afe_control/space_vector ==
  uab_out : Inport
  Bus Creator : BusCreator  Inputs=3
  Bus Selector : BusSelector  OutputSignals=da,db,dc
  Bus Selector1 : BusSelector  OutputSignals=ualpha_ctrl_afe,ubeta_ctrl_afe,ugamma_ctrl_afe
  C Caller : CCaller  FunctionName=sv_pwm_cm_process_simulink  PortSpecificationStruct="%)30     .    B H   8    (     @         %    \"     8    !     0         %  0 \"0    $    _    07)G3F%M90  4&]R=$YA;64 4V-O<&4     26YD97@     5'EP90      4VEZ90      27-';&]B86P   X    P    !@    @    $          4    (     0    ,    !         !   P!O=70 #@   #     &    \"     0         !0    @    !     P    $         $  # &]U=  .    .     8    (    !          %    \"     $    &     0         0   ...(+3252 chars)"
  Constant : Constant  Value=param.glb_time.ts_afe
  Constant1 : Constant
  Data Type Conversion1 : DataTypeConversion  OutDataTypeStr=double  SaturateOnIntegerOverflow=off  RndMeth=Floor
  Data Type Conversion{4,15..16,18} (4 alike) : DataTypeConversion  OutDataTypeStr=single  SaturateOnIntegerOverflow=off  RndMeth=Floor
  Data Type Conversion17 : DataTypeConversion  OutDataTypeStr=uint32  SaturateOnIntegerOverflow=off  RndMeth=Floor
  Data Type Conversion2 : DataTypeConversion  OutDataTypeStr=double  SaturateOnIntegerOverflow=off  RndMeth=Floor
  Data Type Conversion3 : DataTypeConversion  OutDataTypeStr=double  SaturateOnIntegerOverflow=off  RndMeth=Floor
  Gain1 : Gain  Gain=sqrt(3)/2
  Gain2 : Gain  Gain=sqrt(3)/2
  Gain3 : Gain  Gain=param.afe.behav.u_cm_comp_mod1
  duvw : Outport
  wires:
  Data Type Conversion15/1 -> C Caller/2
  Bus Selector/2 -> Data Type Conversion2/1  "<db>"
  Data Type Conversion18/1 -> C Caller/1
  C Caller/1 -> Bus Selector/1
  Bus Creator/1 -> duvw/1
  Data Type Conversion1/1 -> Bus Creator/1  "du(k)"
  Bus Selector1/2 -> Gain2/1  "<ubeta_ctrl_afe>"
  Bus Selector/3 -> Data Type Conversion3/1  "<dc>"
  Bus Selector1/1 -> Gain1/1  "<ualpha_ctrl_afe>"
  Data Type Conversion2/1 -> Bus Creator/2  "dv(k)"
  Gain2/1 -> Data Type Conversion15/1
  Bus Selector/1 -> Data Type Conversion1/1  "<da>"
  Gain1/1 -> Data Type Conversion18/1
  Data Type Conversion3/1 -> Bus Creator/3  "dw(k)"
  Constant/1 -> Data Type Conversion16/1
  uab_out/1 -> Bus Selector1/1
  Constant1/1 -> Data Type Conversion17/1
  Data Type Conversion16/1 -> C Caller/4
  Data Type Conversion17/1 -> C Caller/5
  Bus Selector1/3 -> Gain3/1  "<ugamma_ctrl_afe>"
  Gain3/1 -> Data Type Conversion4/1
  Data Type Conversion4/1 -> C Caller/3

== system afe_dq_ttype/afe_dq_mod1/AFE_control/afe_control/udc_ctrl ==
  udc_pu : Inport
  1/Ti : Gain  Gain=param.afe.ctrl.kp_udc  SaturateOnIntegerOverflow=on  OutDataTypeStr=Inherit: Same as input  ParamDataTypeStr=Inherit: Same as input
  Saturation : Saturate  UpperLimit=param.afe.ctrl.i_ref_lim  LowerLimit=-param.afe.ctrl.i_ref_lim
  Sum1 : Sum  Inputs=+++  SaturateOnIntegerOverflow=on
  Sum2 : Sum  Inputs=-+  SaturateOnIntegerOverflow=on
  Sum3 : Sum  Inputs=-+  SaturateOnIntegerOverflow=on
  To Workspace1 : ToWorkspace  VariableName=udc_pu_sim_mod1  SampleTime=-1
      settings: MaxDataPoints=param.glb_time.Ns_afe
  To Workspace3 : ToWorkspace  VariableName=udc_pu_ref_sim_mod1  SampleTime=-1
      settings: MaxDataPoints=param.glb_time.Ns_afe
  Unit Delay4 : UnitDelay  SampleTime=-1
  discrete-time-low-pass-filter1 : discrete_time_low_pass_filter/discrete-time-low-pass-filter  tau=20e-3  ts=param.glb_time.ts_afe
  kp : Gain  Gain=param.afe.ctrl.ki_udc*param.glb_time.ts_afe  SaturateOnIntegerOverflow=on  OutDataTypeStr=Inherit: Same as input  ParamDataTypeStr=Inherit: Same as input
  udc_norm_ref : Step  Time=1e-3  FinalValue=param.afe.ctrl.udc_pu_ref
  udc_tracking : Scope  NumInputPorts=3
      settings: ActiveDisplayYMinimum=-0.20844726562499993  ActiveDisplayYMaximum=1.856494140625  DataLoggingVariableName=ScopeData8
  i_xi_ref : Outport
  wires:
  1/Ti/1 -> Sum1/1, Sum3/1
  kp/1 -> Sum1/2
  Sum3/1 -> Unit Delay4/1
  Unit Delay4/1 -> Sum1/3
  udc_norm_ref/1 -> discrete-time-low-pass-filter1/1
  udc_pu/1 -> Sum2/1, To Workspace1/1, udc_tracking/2  "udc_pu"
  Sum2/1 -> kp/1, 1/Ti/1
  Sum1/1 -> Saturation/1
  Saturation/1 -> udc_tracking/3, Sum3/2, i_xi_ref/1  "i_xi_ref"
  discrete-time-low-pass-filter1/1 -> To Workspace3/1, udc_tracking/1, Sum2/2  "udc_pu_ref"

== system afe_dq_ttype/afe_dq_mod1/afe/deadtime_generator_for_ttype/dead_time_generator_cmos_simulink_phu ==
  gate_commands : Inport
  Bus Creator : BusCreator  Inputs=4
  Bus Selector : BusSelector  OutputSignals=gate_cmds_phu.cmd_gate_Q1,gate_cmds_phu.cmd_gate_Q4
  Bus Selector1 : BusSelector  OutputSignals=gate_cmds_phu.cmd_gate_Q2,gate_cmds_phu.cmd_gate_Q3
  Transfer Fcn{,1..3} (4 alike) : TransferFcn  Denominator=[ts 1]
  dead_time_leg_generator_1 : Subsystem  mask{Vpos_rail_dtg=positive_voltage_rail, deadtime=dead_time}
      mask prompts: Vpos_rail_dtg "Positive Voltage Rail Supply"; deadtime "DeadTime [s]"
  cmd_gates : Outport
  wires:
  Transfer Fcn1/1 -> dead_time_leg_generator_1/2(cmd_in_QB)  "gate_cmd_Q4"
  Transfer Fcn/1 -> dead_time_leg_generator_1/1(cmd_in_QA)  "gate_cmd_Q1"
  gate_commands/1 -> Bus Selector1/1, Bus Selector/1
  Bus Selector/1 -> Transfer Fcn/1  "<cmd_gate_Q1>"
  Bus Selector/2 -> Transfer Fcn1/1  "<cmd_gate_Q4>"
  Bus Selector1/1 -> Transfer Fcn2/1  "<cmd_gate_Q2>"
  Bus Selector1/2 -> Transfer Fcn3/1  "<cmd_gate_Q3>"
  dead_time_leg_generator_1/1(cmd_out_QA) -> [cmd_gate_Q1]  "cmd_gate_Q1"
  [cmd_gate_Q1] -> Bus Creator/1  "cmd_gate_Q1"
  Bus Creator/1 -> cmd_gates/1
  dead_time_leg_generator_1/2(cmd_out_QB) -> [cmd_gate_Q4]  "cmd_gate_Q4"
  Transfer Fcn3/1 -> [cmd_gate_Q3]  "cmd_gate_Q3"
  Transfer Fcn2/1 -> [cmd_gate_Q2]  "cmd_gate_Q2"
  [cmd_gate_Q2] -> Bus Creator/2  "cmd_gate_Q2"
  [cmd_gate_Q4] -> Bus Creator/4  "cmd_gate_Q4"
  [cmd_gate_Q3] -> Bus Creator/3  "cmd_gate_Q3"

== system afe_dq_ttype/afe_dq_mod1/afe/deadtime_generator_for_ttype/dead_time_generator_cmos_simulink_phv ==
  gate_commands : Inport
  Bus Creator : BusCreator  Inputs=4
  Bus Selector : BusSelector  OutputSignals=gate_cmds_phv.cmd_gate_Q1,gate_cmds_phv.cmd_gate_Q4
  Bus Selector1 : BusSelector  OutputSignals=gate_cmds_phv.cmd_gate_Q2,gate_cmds_phv.cmd_gate_Q3
  Transfer Fcn{,1..3} (4 alike) : TransferFcn  Denominator=[ts 1]
  dead_time_leg_generator_1 : Subsystem  mask{Vpos_rail_dtg=positive_voltage_rail, deadtime=dead_time}
      mask prompts: Vpos_rail_dtg "Positive Voltage Rail Supply"; deadtime "DeadTime [s]"
  cmd_gates : Outport
  wires:
  [cmd_gate_Q3] -> Bus Creator/3  "cmd_gate_Q3"
  [cmd_gate_Q4] -> Bus Creator/4  "cmd_gate_Q4"
  [cmd_gate_Q2] -> Bus Creator/2  "cmd_gate_Q2"
  Transfer Fcn2/1 -> [cmd_gate_Q2]  "cmd_gate_Q2"
  Transfer Fcn3/1 -> [cmd_gate_Q3]  "cmd_gate_Q3"
  dead_time_leg_generator_1/2(cmd_out_QB) -> [cmd_gate_Q4]  "cmd_gate_Q4"
  Bus Creator/1 -> cmd_gates/1
  [cmd_gate_Q1] -> Bus Creator/1  "cmd_gate_Q1"
  dead_time_leg_generator_1/1(cmd_out_QA) -> [cmd_gate_Q1]  "cmd_gate_Q1"
  gate_commands/1 -> Bus Selector1/1, Bus Selector/1
  Transfer Fcn/1 -> dead_time_leg_generator_1/1(cmd_in_QA)  "gate_cmd_Q1"
  Transfer Fcn1/1 -> dead_time_leg_generator_1/2(cmd_in_QB)  "gate_cmd_Q4"
  Bus Selector/1 -> Transfer Fcn/1  "<cmd_gate_Q1>"
  Bus Selector/2 -> Transfer Fcn1/1  "<cmd_gate_Q4>"
  Bus Selector1/1 -> Transfer Fcn2/1  "<cmd_gate_Q2>"
  Bus Selector1/2 -> Transfer Fcn3/1  "<cmd_gate_Q3>"

== system afe_dq_ttype/afe_dq_mod1/afe/deadtime_generator_for_ttype/dead_time_generator_cmos_simulink_phw ==
  gate_commands : Inport
  Bus Creator : BusCreator  Inputs=4
  Bus Selector : BusSelector  OutputSignals=gate_cmds_phw.cmd_gate_Q1,gate_cmds_phw.cmd_gate_Q4
  Bus Selector1 : BusSelector  OutputSignals=gate_cmds_phw.cmd_gate_Q2,gate_cmds_phw.cmd_gate_Q3
  Transfer Fcn{,1..3} (4 alike) : TransferFcn  Denominator=[ts 1]
  dead_time_leg_generator_1 : Subsystem  mask{Vpos_rail_dtg=positive_voltage_rail, deadtime=dead_time}
      mask prompts: Vpos_rail_dtg "Positive Voltage Rail Supply"; deadtime "DeadTime [s]"
  cmd_gates : Outport
  wires:
  Transfer Fcn1/1 -> dead_time_leg_generator_1/2(cmd_in_QB)  "gate_cmd_Q4"
  Transfer Fcn/1 -> dead_time_leg_generator_1/1(cmd_in_QA)  "gate_cmd_Q1"
  gate_commands/1 -> Bus Selector1/1, Bus Selector/1
  dead_time_leg_generator_1/1(cmd_out_QA) -> [cmd_gate_Q1]  "cmd_gate_Q1"
  [cmd_gate_Q1] -> Bus Creator/1  "cmd_gate_Q1"
  Bus Creator/1 -> cmd_gates/1
  dead_time_leg_generator_1/2(cmd_out_QB) -> [cmd_gate_Q4]  "cmd_gate_Q4"
  Transfer Fcn3/1 -> [cmd_gate_Q3]  "cmd_gate_Q3"
  Transfer Fcn2/1 -> [cmd_gate_Q2]  "cmd_gate_Q2"
  [cmd_gate_Q2] -> Bus Creator/2  "cmd_gate_Q2"
  [cmd_gate_Q4] -> Bus Creator/4  "cmd_gate_Q4"
  [cmd_gate_Q3] -> Bus Creator/3  "cmd_gate_Q3"
  Bus Selector/1 -> Transfer Fcn/1  "<cmd_gate_Q1>"
  Bus Selector/2 -> Transfer Fcn1/1  "<cmd_gate_Q4>"
  Bus Selector1/1 -> Transfer Fcn2/1  "<cmd_gate_Q2>"
  Bus Selector1/2 -> Transfer Fcn3/1  "<cmd_gate_Q3>"
